simulink model "sm_car"  (R2025a)
settings: Solver=ode23t  StartTime=0.0  StopTime=400  MaxStep=0.4  RelTol=1e-3  AbsTol=1e-3  EnableMultiTasking=on
PreLoadFcn:
  | % Due to usability issue in Repeating Sequence block
  | warning('off','Simulink:Masking:Invalid');
  | 
  | % Eliminate unnecessary warnings in inactive variants
  | % Warnings generated only if you click through inactive variant
  | warning('off','MATLAB:nonExistentField');
  | warning('off','Simulink:Parameters:BlkParamUndefined');
PostLoadFcn:
  | set_param([bdroot '/Vehicle'],'popup_trailer','Off')
  | warning('off','sm:sli:setup:compile:LocalSolverNotSupported')
  | %sm_car_config_maneuver(bdroot,'WOT Braking');
  | sm_car_config_vehicle(bdroot,'false');
  | sm_car_config_logging(bdroot);
InitFcn:
  | sm_car_config_camera;
  | Vehicle = sm_car_vehcfg_checkConfig(Vehicle);
  | sm_car_check_tire_model(bdroot);
StartFcn:
  | tic;
StopFcn:
  | Elapsed_Sim_Time = toc;
  | % disp(['Elapsed Sim Time = ' num2str(Elapsed_Sim_Time)]);
undefined symbols (not defined in the file): Axle1D, AxleIn, Camera, Control, Driver, Free, Init, Maneuver, Pedal, RaceFix, RaceSpin, Scene, ShaftL1, ShaftL2, ShaftR1, ShaftR2, Soft, Stiff, Visual, X, xy_data_car_side, Y, Z
libraries: sm_lib x1546, nesl_utility x528, fl_lib x480, SimscapeFluids_lib x61, sdl_lib x49, simulink x29, ee_lib x7, simulink_extras x6, Linkage_Systems x4, Tire_1x2x x4, AntiRollBar_Systems x2, Linkage_Decoupled x2
(part 19 of 79)

== system sm_car/Vehicle/Vehicle/Chassis/SuspA1/Linkage/Steer ==
  DrvBus : Inport
  CtrlBus : Inport  Port=2
  Wheel Driven Rack 1UJoint : Subsystem  Tag=PublishSubsystem  VariantControl=WheelDrivenRack1UJoint  mask(Steering System with Wheel Actuation){hp_wheel=Steer.Wheel.sMount.Value, wheel_axis_incl=Steer.Wheel.aAxis.Value, hp_mt_rack=Steer.Rack.sMount.Value, hp_out_rack=Steer.Rack.sOutboard.Value, hp_pinion=Steer.Pinion.sMount.Value, Wheel=Steer.Wheel, len_sha_u=Steer.Shaft_Upper.xLength.Value, sha_u_mass=Steer.Shaft_Upper.m.Value, sha_l_mass=Steer.Shaft_Lower.m.Value, rad_pinion=Steer.Pinion.xRad.Value, pinion_mass=Steer.Pinion.m.Value, rack_mass=Steer.Rack.m.Value, whl2steer_filter=1/Steer.Rack.fActuatorCutoff.Value, clr_rack=Visual.SteeringRack.clr, opc_rack=Visual.part.opc, radius_rack=Visual.SteeringRack.rad, clr_shaft=Visual.SteeringShafts.clr, opc_shaft=Visual.part.opc, size_shaft=Visual.SteeringShafts.rad, clr_pinion=Visual.SteeringPinion.clr, opc_pinion=Visual.part.opc, len_pinion=Visual.SteeringPinion.len, clr_connhp=Visual.hp.clr, opc_connhp=Visual.hp.opc, size_connhp=Visual.hp.rad, clr_wheel=Visual.SteeringWheel.clr, opc_wheel=Visual.part.opc, DriverHuman=Steer.DriverHuman}
      mask prompts: hp_wheel "HP Wheel [xyz] (m)"; wheel_axis_incl "Wheel Axis Angle (rad)"; hp_mt_rack "HP Rack Mount [xyz] (m)"; hp_out_rack "HP Track Rod Inboard [xyz] (m)"; hp_pinion "HP Pinion [xyz] (m)"; whl2steer_filter "Steer Motion Filter (sec)"; DriverHuman "Driver Human (structure)"
      mask help: Actuation is applied to steering wheel and transmitted to rack via shafts in steering column. Assumes constant gear ratio between pinion and rack.
      mask init:
      | % Calculate inclination of pinion gear about rack travel axis
      | pinion_incl = atan2(hp_mt_rack(1)-hp_pinion(1),hp_mt_rack(3)-hp_pinion(3));
      | 
      | % Calculate location of universal joint
      | hp_col_upper = hp_wheel  + [+len_sha_u*cos(wheel_axis_incl)  0 -len_sha_u*sin(wheel_axis_incl)];
      mask TypeOptions hp_wheel:
      | Ref to Wheel/Transform
      | HP Wheel/TranslationCartesianOffset
      mask TypeOptions hp_mt_rack:
      | Ref to Rack/Transform
      | HP Rack/TranslationCartesianOffset
      mask TypeOptions hp_out_rack: Rack/hp_out
      mask TypeOptions rack_mass: Rack/rack_mass
      mask TypeOptions whl2steer_filter: Physical Signal/InputFilterTimeConstant
      mask TypeOptions clr_rack: Rack/clr_rack
      mask TypeOptions opc_rack: Rack/opc_rack
      mask TypeOptions radius_rack: Rack/radius_rack
      mask TypeOptions clr_shaft:
      | Shaft
      | Steering/Shaft/GraphicDiffuseColor | Shaft
      | Lower/Shaft/GraphicDiffuseColor | Shaft
      | Intermediate/Shaft/GraphicDiffuseColor
      mask TypeOptions opc_shaft:
      | Shaft
      | Steering/Shaft/GraphicOpacity | Shaft
      | Lower/Shaft/GraphicOpacity | Shaft
      | Intermediate/Shaft/GraphicOpacity
      mask TypeOptions size_shaft:
      | Shaft
      | Steering/Shaft/CylinderRadius | Shaft
      | Lower/Shaft/CylinderRadius | Shaft
      | Intermediate/Shaft/CylinderRadius
      mask TypeOptions clr_pinion: Pinion/Pinion/GraphicDiffuseColor
      mask TypeOptions opc_pinion: Pinion/Pinion/GraphicOpacity
      mask TypeOptions len_pinion: Pinion/Pinion/CylinderLength
      mask TypeOptions clr_connhp:
      | Ref to Rack/Vis
      | Rack
      | Housing/GraphicDiffuseColor | HPs/HP Lower Col/GraphicDiffuseColor | HPs/HP Pinion/GraphicDiffuseColor | HPs/HP Upper Col/GraphicDiffuseColor
      mask TypeOptions opc_connhp:
      | Ref to Rack/Vis
      | Rack
      | Housing/GraphicOpacity | HPs/HP Lower Col/GraphicOpacity | HPs/HP Pinion/GraphicOpacity | HPs/HP Upper Col/GraphicOpacity
      mask TypeOptions size_connhp:
      | Ref to Rack/Vis
      | Rack
      | Housing/SphereRadius | HPs/HP Lower Col/SphereRadius | HPs/HP Pinion/SphereRadius | HPs/HP Upper Col/SphereRadius
      mask TypeOptions clr_wheel: Wheel/clr_wheel
      mask TypeOptions opc_wheel: Wheel/opc_wheel
      mask DialogControl cont_steer Prompt: Steer
      mask DialogControl grp_strparts Prompt: Parts
      mask DialogControl text_strparts_len Prompt: Length/Radius (m)
      mask DialogControl text_strparts_mass Prompt: Mass (kg)
      mask DialogControl text_strparts_wheel Prompt: Wheel
      mask DialogControl text_strparts_wheel_m Prompt: <CAD file>
      mask DialogControl text_strparts_sha_u Prompt: Upper Shaft
      mask DialogControl text_strparts_sha_i Prompt: Lower Shaft
      mask DialogControl text_strparts_sha_i_len Prompt: <length upper, lower>
      mask DialogControl text_strparts_pinion Prompt: Pinion
      mask DialogControl text_strparts_rack Prompt: Rack
      mask DialogControl text_strparts_rack_len Prompt: <HP Rod Inboard>
      mask DialogControl grp_steering Prompt: Steering Input
      mask DialogControl cont_vis_steer Prompt: Visualization
      mask DialogControl text_steer_vis_clr Prompt: Color [RGB]
      mask DialogControl text_steer_vis_opc Prompt: Opac. (0-1)
      mask DialogControl text_steer_vis_size Prompt: Size (m)
      mask DialogControl text_steer_vis_rack Prompt: Rack
      mask DialogControl text_steer_vis_shafts Prompt: Shafts
      mask DialogControl text_steer_vis_pinion Prompt: Pinion
      mask DialogControl text_steer_vis_connhp Prompt: Connections, HP
      mask DialogControl text_steer_vis_wheel Prompt: Wheel
      mask DialogControl text_steer_size_wheel Prompt: <CAD File>
      mask DialogControl cont_driver_human Prompt: Driver Human
  " rodL" : PMIOPort  Side=Right
  " ref" : PMIOPort  Port=2  Side=Right
  " rodR" : PMIOPort  Port=3  Side=Right
  " meas" : Outport  VectorParamsAs1DForOutWhenUnconnected=off

== system sm_car/Vehicle/Vehicle/Chassis/SuspA1/Linkage/Wheel Meas Left ==
  note: For Steering Axis Inclination Estimation
  Bus Creator : BusCreator  Inputs=4
  Calculate Camber : Subsystem
  Calculate Camber Z Axis : Subsystem
  Calculate Toe : Subsystem
  Calculate Toe X Axis : Subsystem
  PS-Simulink Converter1 : nesl_utility/PS-Simulink Converter  PhysicalDomain=network_engine_domain  SubClassName=ps_output  LeftPortType=input  RightPortType=output  PseudoPeriodic=off  Frequencies=[]  VectorFormat=1-D array  Unit=1  AffineConversion=off
  Select x axis : Selector  NumberOfDimensions=2  InputPortWidth=2  IndexOptions=Index vector (dialog),Index vector (dialog)  Indices=[1 2 3],1  OutputSizes=1,1
  Select z axis : Selector  NumberOfDimensions=2  InputPortWidth=2  IndexOptions=Index vector (dialog),Index vector (dialog)  Indices=[1 2 3],3  OutputSizes=1,1
  Sign LR aCamber : Gain  Gain=180/pi*rhs_tc
  Sign LR aCamberX : Gain  Gain=180/pi*rhs_tc
  Sign LR aToe : Gain  Gain=180/pi*rhs_tc
  Sign LR aToeX : Gain  Gain=180/pi*rhs_tc
  Transform Sensor : sm_lib/Frames and Transforms/Transform Sensor  MeasurementFrame=Base  RotationSequence=XYX  SenseAngle=off  SenseAxis=off  SenseQ=off  SenseR=on  SenseRotationSequence=off  SenseOmegaX=off  SenseOmegaY=off  SenseOmegaZ=off  SenseOmega=off  SenseQDot=off  SenseRDot=off  SenseRotationSequenceDot=off  SenseAlphaX=off  SenseAlphaY=off  SenseAlphaZ=off  SenseAlpha=off  SenseQDDot=off  SenseRDDot=off  SenseX=off  SenseY=off  SenseZ=off  SenseXYZ=off  SenseRad=off  SenseAzim=off  SenseDist=off  SenseInc=off  SenseXDot=off  SenseYDot=off  SenseZDot=off  SenseXYZDot=off  SenseRadDot=off  SenseAzimDot=off  SenseDistDot=off  SenseIncDot=off  SenseXDDot=off  SenseYDDot=off  SenseZDDot=off  SenseXYZDDot=off  SenseRadDDot=off  SenseAzimDDot=off  SenseDistDDot=off  SenseIncDDot=off
  Ref : PMIOPort  Side=Left
  Whl Ctr : PMIOPort  Port=2  Side=Left
  meas : Outport  VectorParamsAs1DForOutWhenUnconnected=off
  wires:
  Calculate Toe X Axis/1(Toe) -> Sign LR aToeX/1
  Calculate Camber Z Axis/1(Camber) -> Sign LR aCamberX/1
  Sign LR aCamberX/1 -> Bus Creator/4  "aCamberX"
  Select x axis/1 -> Calculate Toe X Axis/1(uvec spin axis), Calculate Camber Z Axis/1(uvec spin axis)
  Sign LR aToeX/1 -> Bus Creator/3  "aToeX"
  Bus Creator/1 -> meas/1  "Whl"
  Sign LR aToe/1 -> Bus Creator/1  "aToe"
  Sign LR aCamber/1 -> Bus Creator/2  "aCamber"
  PS-Simulink Converter1/1 -> Select x axis/1, Select z axis/1
  Select z axis/1 -> Calculate Camber/1(uvec spin axis), Calculate Toe/1(uvec spin axis)  "uvec spin axis"
  Calculate Camber/1(Camber) -> Sign LR aCamber/1
  Calculate Toe/1(Toe) -> Sign LR aToe/1
  connections:
  Transform Sensor/LConn1 -- Ref/RConn1
  Transform Sensor/RConn1 -- Whl Ctr/RConn1
  PS-Simulink Converter1/LConn1 -- Transform Sensor/RConn2

== system sm_car/Vehicle/Vehicle/Chassis/SuspA1/Linkage/Wheel Meas Right ==
  note: For Steering Axis Inclination Estimation
  Bus Creator : BusCreator  Inputs=4
  Calculate Camber : Subsystem
  Calculate Camber Z Axis : Subsystem
  Calculate Toe : Subsystem
  Calculate Toe X Axis : Subsystem
  PS-Simulink Converter1 : nesl_utility/PS-Simulink Converter  PhysicalDomain=network_engine_domain  SubClassName=ps_output  LeftPortType=input  RightPortType=output  PseudoPeriodic=off  Frequencies=[]  VectorFormat=1-D array  Unit=1  AffineConversion=off
  Select x axis : Selector  NumberOfDimensions=2  InputPortWidth=2  IndexOptions=Index vector (dialog),Index vector (dialog)  Indices=[1 2 3],1  OutputSizes=1,1
  Select z axis : Selector  NumberOfDimensions=2  InputPortWidth=2  IndexOptions=Index vector (dialog),Index vector (dialog)  Indices=[1 2 3],3  OutputSizes=1,1
  Sign LR aCamber : Gain  Gain=180/pi*rhs_tc
  Sign LR aCamberX : Gain  Gain=180/pi*rhs_tc
  Sign LR aToe : Gain  Gain=180/pi*rhs_tc
  Sign LR aToeX : Gain  Gain=180/pi*rhs_tc
  Transform Sensor : sm_lib/Frames and Transforms/Transform Sensor  MeasurementFrame=Base  RotationSequence=XYX  SenseAngle=off  SenseAxis=off  SenseQ=off  SenseR=on  SenseRotationSequence=off  SenseOmegaX=off  SenseOmegaY=off  SenseOmegaZ=off  SenseOmega=off  SenseQDot=off  SenseRDot=off  SenseRotationSequenceDot=off  SenseAlphaX=off  SenseAlphaY=off  SenseAlphaZ=off  SenseAlpha=off  SenseQDDot=off  SenseRDDot=off  SenseX=off  SenseY=off  SenseZ=off  SenseXYZ=off  SenseRad=off  SenseAzim=off  SenseDist=off  SenseInc=off  SenseXDot=off  SenseYDot=off  SenseZDot=off  SenseXYZDot=off  SenseRadDot=off  SenseAzimDot=off  SenseDistDot=off  SenseIncDot=off  SenseXDDot=off  SenseYDDot=off  SenseZDDot=off  SenseXYZDDot=off  SenseRadDDot=off  SenseAzimDDot=off  SenseDistDDot=off  SenseIncDDot=off
  Ref : PMIOPort  Side=Left
  Whl Ctr : PMIOPort  Port=2  Side=Left
  meas : Outport  VectorParamsAs1DForOutWhenUnconnected=off
  wires:
  Calculate Toe X Axis/1(Toe) -> Sign LR aToeX/1
  Calculate Camber Z Axis/1(Camber) -> Sign LR aCamberX/1
  Sign LR aCamberX/1 -> Bus Creator/4  "aCamberX"
  Select x axis/1 -> Calculate Toe X Axis/1(uvec spin axis), Calculate Camber Z Axis/1(uvec spin axis)
  Sign LR aToeX/1 -> Bus Creator/3  "aToeX"
  Bus Creator/1 -> meas/1  "Whl"
  Sign LR aToe/1 -> Bus Creator/1  "aToe"
  Sign LR aCamber/1 -> Bus Creator/2  "aCamber"
  PS-Simulink Converter1/1 -> Select x axis/1, Select z axis/1
  Select z axis/1 -> Calculate Camber/1(uvec spin axis), Calculate Toe/1(uvec spin axis)  "uvec spin axis"
  Calculate Camber/1(Camber) -> Sign LR aCamber/1
  Calculate Toe/1(Toe) -> Sign LR aToe/1
  connections:
  Transform Sensor/LConn1 -- Ref/RConn1
  Transform Sensor/RConn1 -- Whl Ctr/RConn1
  PS-Simulink Converter1/LConn1 -- Transform Sensor/RConn2

== system sm_car/Vehicle/Vehicle/Chassis/SuspA1/Linkage Decoupled/RollHeave Decouple ==
  HP Heave L : Subsystem  mask(Revolute Joint 3 Points){popup_leftRight=Left, hp_bcr_pivot=hp_bcr_pivot, hp_pushrod_in=hp_pushrod, hp_bcr_shock=hp_bcr_shock_heaveL}
      mask prompts: popup_leftRight "Left/Right"; hp_bcr_pivot "HP Bellcrank Pivot [xyz] (m)"; hp_pushrod_in "HP Pushrod Inner [xyz] (m)"; hp_bcr_shock "HP Bellcrank Shock Heave [xyz] (m)"
      mask help: Revolute Joint with degree of freedom normal to 3 hardpoints.
      mask init:
      | % Set parameter for mirroring (+y or -y)
      | if(popup_leftRight == 1)
      |     rhs_susp = 1;    
      | elseif(popup_leftRight == 2)
      |     rhs_susp = -1;
      | end
      | 
      | rhs_hp = [1 rhs_susp 1];
      mask TypeOptions popup_leftRight: Left | Right
      mask Display: image('sm_car_variant_revolute.png')
  HP HeaveR : Subsystem  mask(Revolute Joint 3 Points){popup_leftRight=Right, hp_bcr_pivot=hp_bcr_pivot, hp_pushrod_in=hp_pushrod, hp_bcr_shock=hp_bcr_shock_heaveR}
      mask prompts: popup_leftRight "Left/Right"; hp_bcr_pivot "HP Bellcrank Pivot [xyz] (m)"; hp_pushrod_in "HP Pushrod Inner [xyz] (m)"; hp_bcr_shock "HP Bellcrank Shock Heave [xyz] (m)"
      mask help: Revolute Joint with degree of freedom normal to 3 hardpoints.
      mask init:
      | % Set parameter for mirroring (+y or -y)
      | if(popup_leftRight == 1)
      |     rhs_susp = 1;    
      | elseif(popup_leftRight == 2)
      |     rhs_susp = -1;
      | end
      | 
      | rhs_hp = [1 rhs_susp 1];
      mask TypeOptions popup_leftRight: Left | Right
      mask Display: image('sm_car_variant_revolute.png')
  HP Roll L : Subsystem  mask(Revolute Joint 3 Points){popup_leftRight=Left, hp_bcr_pivot=hp_bcr_pivot, hp_pushrod_in=hp_pushrod, hp_bcr_shock=hp_bcr_shock_heaveL}
      mask prompts: popup_leftRight "Left/Right"; hp_bcr_pivot "HP Bellcrank Pivot [xyz] (m)"; hp_pushrod_in "HP Pushrod Inner [xyz] (m)"; hp_bcr_shock "HP Bellcrank Shock Heave [xyz] (m)"
      mask help: Revolute Joint with degree of freedom normal to 3 hardpoints.
      mask init:
      | % Set parameter for mirroring (+y or -y)
      | if(popup_leftRight == 1)
      |     rhs_susp = 1;    
      | elseif(popup_leftRight == 2)
      |     rhs_susp = -1;
      | end
      | 
      | rhs_hp = [1 rhs_susp 1];
      mask TypeOptions popup_leftRight: Left | Right
      mask Display: image('sm_car_variant_revolute.png')
  HP Roll R : Subsystem  mask(Revolute Joint 3 Points){popup_leftRight=Right, hp_bcr_pivot=hp_bcr_pivot, hp_pushrod_in=hp_pushrod, hp_bcr_shock=hp_bcr_shock_heaveR}
      mask prompts: popup_leftRight "Left/Right"; hp_bcr_pivot "HP Bellcrank Pivot [xyz] (m)"; hp_pushrod_in "HP Pushrod Inner [xyz] (m)"; hp_bcr_shock "HP Bellcrank Shock Heave [xyz] (m)"
      mask help: Revolute Joint with degree of freedom normal to 3 hardpoints.
      mask init:
      | % Set parameter for mirroring (+y or -y)
      | if(popup_leftRight == 1)
      |     rhs_susp = 1;    
      | elseif(popup_leftRight == 2)
      |     rhs_susp = -1;
      | end
      | 
      | rhs_hp = [1 rhs_susp 1];
      mask TypeOptions popup_leftRight: Left | Right
      mask Display: image('sm_car_variant_revolute.png')
  PS-Simulink Converter{,1..3} (4 alike) : nesl_utility/PS-Simulink Converter  PhysicalDomain=network_engine_domain  SubClassName=ps_output  LeftPortType=input  RightPortType=output  PseudoPeriodic=off  Frequencies=[]  VectorFormat=1-D array  Unit=1  AffineConversion=off
  Shock Heave : Subsystem  mask{shock_pist_mass=shock_pist_mass_heave, shock_cyl_mass=shock_cyl_mass_heave, hp_spr_top=hp_bcr_shock_heaveR, hp_spr_bot=hp_bcr_shock_heaveL, up_lim_bumpstop=up_lim_bumpstop_heave, low_lim_bumpstop=low_lim_bumpstop_heave, clr_conn_shock=clr_conn_shock, opc_conn_shock=opc_conn_shock, size_conn_shock=size_conn_shock, clr_shock_cyl=clr_shock_cyl, opc_shock_cyl=opc_shock_cyl, radius_shock_cyl=radius_shock_cyl, clr_shock_piston=clr_shock_piston, opc_shock_piston=opc_shock_piston, clr_shock_bumpstop=clr_shock_bumpstop, opc_shock_bumpstop=opc_shock_bumpstop, deadvol_len_shock_cyl=deadvol_len_shock_cyl, piston_len_shock=piston_len_shock, cyl_cap_len_shock=cyl_cap_len_shock, bumpstop_len_shock=bumpstop_len_shock}
      mask prompts: shock_pist_mass "Piston Mass (kg)"; shock_cyl_mass "Cylinder Mass (kg)"; hp_spr_top "Shock Top [xyz] (m)"; hp_spr_bot "Shock Bottom [xyz] (m)"; up_lim_bumpstop "Upper Limit Bumpstop (m)"; low_lim_bumpstop "Lower Limit Bumpstop (m)"; deadvol_len_shock_cyl "Dead Volume Height (m)"; piston_len_shock "Piston Length (m)"; cyl_cap_len_shock "Cylinder Cap Length (m)"; bumpstop_len_shock "Bumpstop Length (m)"
      mask init:
      | init_spr_len = norm(hp_spr_top-hp_spr_bot);
      | 
      | rod_length_upper = ...
      | cyl_cap_len_shock + bumpstop_len_shock + abs(low_lim_bumpstop) + ...
      | cyl_cap_len_shock + abs(up_lim_bumpstop) + piston_len_shock;
      | 
      | rod_length_lower = init_spr_len - rod_length_upper - deadvol_len_shock_cyl - cyl_cap_len_shock - abs(low_lim_bumpstop);
      | 
      | bumpstop_xc_rev = [0 0; 0.7 0; 0.9 1; 0 1].*[radius_shock_cyl bumpstop_len_shock];
      | 
      | cyl_wall_length = piston_len_shock+abs(low_lim_bumpstop)+abs(up_lim_bumpstop)+deadvol_len_shock_cyl;
      mask Help: web('sm_car_doc_susp_shock.html')
      mask TypeOptions shock_pist_mass: Piston/Rod/Mass
      mask TypeOptions shock_cyl_mass: Cylinder/Wall/Mass
      mask TypeOptions clr_conn_shock:
      | Vis
      | HP L/GraphicDiffuseColor | Vis
      | HP U/GraphicDiffuseColor
      mask TypeOptions opc_conn_shock:
      | Vis
      | HP L/GraphicOpacity | Vis
      | HP U/GraphicOpacity
      mask TypeOptions clr_shock_cyl: Cylinder/Cap Bottom/GraphicDiffuseColor | Cylinder/Cap Top/GraphicDiffuseColor | Cylinder/Wall/GraphicDiffuseColor
      mask TypeOptions clr_shock_piston: Piston/Cap/GraphicDiffuseColor | Piston/Piston/GraphicDiffuseColor | Piston/Rod/GraphicDiffuseColor
      mask TypeOptions opc_shock_piston: Piston/Cap/GraphicOpacity | Piston/Piston/GraphicOpacity | Piston/Rod/GraphicOpacity
      mask TypeOptions clr_shock_bumpstop: Piston/Bumpstop/GraphicDiffuseColor
      mask TypeOptions opc_shock_bumpstop: Piston/Bumpstop/GraphicOpacity
      mask DialogControl cont_shock Prompt: Shock
      mask DialogControl cont_vis_shock Prompt: Visualization
      mask DialogControl text_blank_shock Prompt: (Add text here)
      mask DialogControl text_clr_shock Prompt: Color  [RGB]
      mask DialogControl text_opc_shock Prompt: Opac. (0-1)
      mask DialogControl text_size_shock Prompt: Size (m)
      mask DialogControl text_conn_shock Prompt: Connections
      mask DialogControl text_shock_cyl Prompt: Cylinder
      mask DialogControl text_shock_piston Prompt: Piston
      mask DialogControl text_piston_radius Prompt: <cylinder radius>
      mask DialogControl text_shock_bumpstop Prompt: Bumpstop
      mask DialogControl text_bumpstop_radius Prompt: <cylinder radius>
      mask Display: image('sm_car_vehicle_linkage_shock_hpu_IMAGE.png');
  Shock Roll : Subsystem  mask{shock_pist_mass=shock_pist_mass_roll, shock_cyl_mass=shock_cyl_mass_roll, hp_spr_top=hp_bcr_shock_rollR, hp_spr_bot=hp_bcr_shock_rollL, up_lim_bumpstop=up_lim_bumpstop_roll, low_lim_bumpstop=low_lim_bumpstop_roll, clr_conn_shock=clr_conn_shock, opc_conn_shock=opc_conn_shock, size_conn_shock=size_conn_shock, clr_shock_cyl=clr_shock_cyl, opc_shock_cyl=opc_shock_cyl, radius_shock_cyl=radius_shock_cyl, clr_shock_piston=clr_shock_piston, opc_shock_piston=opc_shock_piston, clr_shock_bumpstop=clr_shock_bumpstop, opc_shock_bumpstop=opc_shock_bumpstop, deadvol_len_shock_cyl=deadvol_len_shock_cyl, piston_len_shock=piston_len_shock, cyl_cap_len_shock=cyl_cap_len_shock, bumpstop_len_shock=bumpstop_len_shock}
      mask prompts: shock_pist_mass "Piston Mass (kg)"; shock_cyl_mass "Cylinder Mass (kg)"; hp_spr_top "Shock Top [xyz] (m)"; hp_spr_bot "Shock Bottom [xyz] (m)"; up_lim_bumpstop "Upper Limit Bumpstop (m)"; low_lim_bumpstop "Lower Limit Bumpstop (m)"; deadvol_len_shock_cyl "Dead Volume Height (m)"; piston_len_shock "Piston Length (m)"; cyl_cap_len_shock "Cylinder Cap Length (m)"; bumpstop_len_shock "Bumpstop Length (m)"
      mask init: same as sm_car/Vehicle/Vehicle/Chassis/SuspA1/Linkage Decoupled/RollHeave Decouple/Shock Heave
      mask Help: web('sm_car_doc_susp_shock.html')
      mask TypeOptions shock_pist_mass: Piston/Rod/Mass
      mask TypeOptions shock_cyl_mass: Cylinder/Wall/Mass
      mask TypeOptions clr_conn_shock:
      | Vis
      | HP L/GraphicDiffuseColor | Vis
      | HP U/GraphicDiffuseColor
      mask TypeOptions opc_conn_shock:
      | Vis
      | HP L/GraphicOpacity | Vis
      | HP U/GraphicOpacity
      mask TypeOptions clr_shock_cyl: Cylinder/Cap Bottom/GraphicDiffuseColor | Cylinder/Cap Top/GraphicDiffuseColor | Cylinder/Wall/GraphicDiffuseColor
      mask TypeOptions clr_shock_piston: Piston/Cap/GraphicDiffuseColor | Piston/Piston/GraphicDiffuseColor | Piston/Rod/GraphicDiffuseColor
      mask TypeOptions opc_shock_piston: Piston/Cap/GraphicOpacity | Piston/Piston/GraphicOpacity | Piston/Rod/GraphicOpacity
      mask TypeOptions clr_shock_bumpstop: Piston/Bumpstop/GraphicDiffuseColor
      mask TypeOptions opc_shock_bumpstop: Piston/Bumpstop/GraphicOpacity
      mask DialogControl cont_shock Prompt: Shock
      mask DialogControl cont_vis_shock Prompt: Visualization
      mask DialogControl text_blank_shock Prompt: (Add text here)
      mask DialogControl text_clr_shock Prompt: Color  [RGB]
      mask DialogControl text_opc_shock Prompt: Opac. (0-1)
      mask DialogControl text_size_shock Prompt: Size (m)
      mask DialogControl text_conn_shock Prompt: Connections
      mask DialogControl text_shock_cyl Prompt: Cylinder
      mask DialogControl text_shock_piston Prompt: Piston
      mask DialogControl text_piston_radius Prompt: <cylinder radius>
      mask DialogControl text_shock_bumpstop Prompt: Bumpstop
      mask DialogControl text_bumpstop_radius Prompt: <cylinder radius>
      mask Display: image('sm_car_vehicle_linkage_shock_hpu_IMAGE.png');
  Transform Align Axis 2P HeaveL : Subsystem  mask(Transform Align Axis Two Points){hp_b=hp_bcr_shock_heaveL, hp_t=hp_bcr_shock_heaveR, popup_f_axis=+Z}
      mask prompts: hp_b "Location of B [xyz] (m)"; hp_t "Target for Frame Axis [xyz] (m)"; popup_f_axis "Axis of F Frame to Aim at Target"
      mask help: Transforms a frame to aim a selected axis at a target point. Both points must be defined relative to the same reference frame.
      mask init:
      | switch popup_f_axis
      |     case 1, vec = [ 1  0  0];
      |     case 2, vec = [ 0  1  0];
      |     case 3, vec = [ 0  0  1];
      |     case 4, vec = [-1  0  0];
      |     case 5, vec = [ 0 -1  0];
      |     case 6, vec = [ 0  0 -1];
      | end
      | 
      | uvec_bt = (hp_t-hp_b)/norm(hp_t-hp_b);
      | rotaxis = cross(vec,uvec_bt);
      | 
      | if (norm(rotaxis)==0)
      |     if (uvec_bt==0)            % hps collocated
      |         rotangle = 0; 
      |     elseif ((uvec_bt+vec)==0)  % vectors antiparallel    
      |         rotangle = pi;
      |         rotaxis = circshift(vec,1);
      |     else                       % vectors parallel
      |         rotangle = 0;          
      |     end
      | else
      |     rotangle = acos(dot(vec,uvec_bt));
      |     %rotangle = acos(dot(vec,(hp_t-hp_b)/norm((hp_t-hp_b))))
      | end
      mask TypeOptions popup_f_axis: +X | +Y | +Z | -X | -Y | -Z
      mask Display: image('sm_car_transform_align_axis_two_points.png')
  Transform Align Axis 2P HeaveR : Subsystem  mask(Transform Align Axis Two Points){hp_b=hp_bcr_shock_heaveR, hp_t=hp_bcr_shock_heaveL, popup_f_axis=-Z}
      mask prompts: hp_b "Location of B [xyz] (m)"; hp_t "Target for Frame Axis [xyz] (m)"; popup_f_axis "Axis of F Frame to Aim at Target"
      mask help: Transforms a frame to aim a selected axis at a target point. Both points must be defined relative to the same reference frame.
      mask init: same as sm_car/Vehicle/Vehicle/Chassis/SuspA1/Linkage Decoupled/RollHeave Decouple/Transform Align Axis 2P HeaveL
      mask TypeOptions popup_f_axis: +X | +Y | +Z | -X | -Y | -Z
      mask Display: image('sm_car_transform_align_axis_two_points.png')
  Transform Align Axis 2P RollL : Subsystem  mask(Transform Align Axis Two Points){hp_b=hp_bcr_shock_rollL, hp_t=hp_bcr_shock_rollR, popup_f_axis=+Z}
      mask prompts: hp_b "Location of B [xyz] (m)"; hp_t "Target for Frame Axis [xyz] (m)"; popup_f_axis "Axis of F Frame to Aim at Target"
      mask help: Transforms a frame to aim a selected axis at a target point. Both points must be defined relative to the same reference frame.
      mask init: same as sm_car/Vehicle/Vehicle/Chassis/SuspA1/Linkage Decoupled/RollHeave Decouple/Transform Align Axis 2P HeaveL
      mask TypeOptions popup_f_axis: +X | +Y | +Z | -X | -Y | -Z
      mask Display: image('sm_car_transform_align_axis_two_points.png')
  Transform Align Axis 2P RollR : Subsystem  mask(Transform Align Axis Two Points){hp_b=hp_bcr_shock_rollR, hp_t=hp_bcr_shock_rollL, popup_f_axis=-Z}
      mask prompts: hp_b "Location of B [xyz] (m)"; hp_t "Target for Frame Axis [xyz] (m)"; popup_f_axis "Axis of F Frame to Aim at Target"
      mask help: Transforms a frame to aim a selected axis at a target point. Both points must be defined relative to the same reference frame.
      mask init: same as sm_car/Vehicle/Vehicle/Chassis/SuspA1/Linkage Decoupled/RollHeave Decouple/Transform Align Axis 2P HeaveL
      mask TypeOptions popup_f_axis: +X | +Y | +Z | -X | -Y | -Z
      mask Display: image('sm_car_transform_align_axis_two_points.png')
  "Transform HP Heave L " : sm_lib/Frames and Transforms/Rigid Transform  RotationMethod=None  FollAlignAxisA=+X  BaseAlignAxisA=+Y  FollAlignAxisB=+Y  BaseAlignAxisB=+Z  RotationStandardAxis=+Z  RotationAngle=0.0  RotationAngleUnits=deg  RotationArbitraryAxis=[0 0 1]  RotationSequenceAxes=FollowerAxes  RotationSequence=XYX  RotationSequenceAngles=[0 0 0]  RotationSequenceAnglesUnits=deg  RotationMatrix=[1 0 0; 0 1 0; 0 0 1]  Quaternion=[1 0 0 0]  TranslationMethod=Cartesian  TranslationCartesianOffset=hp_bcr_shock_heaveL  TranslationCartesianOffsetUnits=m  TranslationStandardAxis=+Z  TranslationStandardOffset=0  TranslationStandardOffsetUnits=m  TranslationROffset=0  TranslationROffsetUnits=m  TranslationThetaOffset=0  TranslationThetaOffsetUnits=deg  TranslationZOffset=0  TranslationZOffsetUnits=m
  Transform HP Heave R : sm_lib/Frames and Transforms/Rigid Transform  RotationMethod=None  FollAlignAxisA=+X  BaseAlignAxisA=+Y  FollAlignAxisB=+Y  BaseAlignAxisB=+Z  RotationStandardAxis=+Z  RotationAngle=0.0  RotationAngleUnits=deg  RotationArbitraryAxis=[0 0 1]  RotationSequenceAxes=FollowerAxes  RotationSequence=XYX  RotationSequenceAngles=[0 0 0]  RotationSequenceAnglesUnits=deg  RotationMatrix=[1 0 0; 0 1 0; 0 0 1]  Quaternion=[1 0 0 0]  TranslationMethod=Cartesian  TranslationCartesianOffset=hp_bcr_shock_heaveR  TranslationCartesianOffsetUnits=m  TranslationStandardAxis=+Z  TranslationStandardOffset=0  TranslationStandardOffsetUnits=m  TranslationROffset=0  TranslationROffsetUnits=m  TranslationThetaOffset=0  TranslationThetaOffsetUnits=deg  TranslationZOffset=0  TranslationZOffsetUnits=m
  Transform HP Roll L : sm_lib/Frames and Transforms/Rigid Transform  RotationMethod=None  FollAlignAxisA=+X  BaseAlignAxisA=+Y  FollAlignAxisB=+Y  BaseAlignAxisB=+Z  RotationStandardAxis=+Z  RotationAngle=0.0  RotationAngleUnits=deg  RotationArbitraryAxis=[0 0 1]  RotationSequenceAxes=FollowerAxes  RotationSequence=XYX  RotationSequenceAngles=[0 0 0]  RotationSequenceAnglesUnits=deg  RotationMatrix=[1 0 0; 0 1 0; 0 0 1]  Quaternion=[1 0 0 0]  TranslationMethod=Cartesian  TranslationCartesianOffset=hp_bcr_shock_rollL  TranslationCartesianOffsetUnits=m  TranslationStandardAxis=+Z  TranslationStandardOffset=0  TranslationStandardOffsetUnits=m  TranslationROffset=0  TranslationROffsetUnits=m  TranslationThetaOffset=0  TranslationThetaOffsetUnits=deg  TranslationZOffset=0  TranslationZOffsetUnits=m
  Transform HP Roll R : sm_lib/Frames and Transforms/Rigid Transform  RotationMethod=None  FollAlignAxisA=+X  BaseAlignAxisA=+Y  FollAlignAxisB=+Y  BaseAlignAxisB=+Z  RotationStandardAxis=+Z  RotationAngle=0.0  RotationAngleUnits=deg  RotationArbitraryAxis=[0 0 1]  RotationSequenceAxes=FollowerAxes  RotationSequence=XYX  RotationSequenceAngles=[0 0 0]  RotationSequenceAnglesUnits=deg  RotationMatrix=[1 0 0; 0 1 0; 0 0 1]  Quaternion=[1 0 0 0]  TranslationMethod=Cartesian  TranslationCartesianOffset=hp_bcr_shock_rollR  TranslationCartesianOffsetUnits=m  TranslationStandardAxis=+Z  TranslationStandardOffset=0  TranslationStandardOffsetUnits=m  TranslationROffset=0  TranslationROffsetUnits=m  TranslationThetaOffset=0  TranslationThetaOffsetUnits=deg  TranslationZOffset=0  TranslationZOffsetUnits=m
  SHL : PMIOPort  Side=Left
  SRL : PMIOPort  Port=2  Side=Left
  SH : PMIOPort  Port=3  Side=Left
  DH : PMIOPort  Port=4  Side=Left
  DR : PMIOPort  Port=5  Side=Left
  SR : PMIOPort  Port=6  Side=Left
  SRR : PMIOPort  Port=7  Side=Left
  SHR : PMIOPort  Port=8  Side=Left
  Out Bus Element : Outport  VectorParamsAs1DForOutWhenUnconnected=off  PortName=meas  Element=qHL
  Out Bus Element3 : Outport  VectorParamsAs1DForOutWhenUnconnected=off  PortName=meas  Element=qHR
  Out Bus Element1 : Outport  VectorParamsAs1DForOutWhenUnconnected=off  PortName=meas  Element=qRL
  Out Bus Element2 : Outport  VectorParamsAs1DForOutWhenUnconnected=off  PortName=meas  Element=qRR
  Out Bus Element4 : Outport  VectorParamsAs1DForOutWhenUnconnected=off  PortName=meas  Element=xHeave
  Out Bus Element5 : Outport  VectorParamsAs1DForOutWhenUnconnected=off  PortName=meas  Element=xRoll
  wires:
  Shock Roll/1(m) -> Out Bus Element5/1
  Shock Heave/1(m) -> Out Bus Element4/1
  PS-Simulink Converter3/1 -> Out Bus Element2/1
  PS-Simulink Converter2/1 -> Out Bus Element3/1
  PS-Simulink Converter1/1 -> Out Bus Element/1
  PS-Simulink Converter/1 -> Out Bus Element1/1
  connections:
  PS-Simulink Converter3/LConn1 -- HP Roll R/RConn2
  PS-Simulink Converter2/LConn1 -- HP HeaveR/RConn2
  PS-Simulink Converter1/LConn1 -- HP Heave L/RConn2
  PS-Simulink Converter/LConn1 -- HP Roll L/RConn2
  HP Heave L/RConn1 -- Transform Align Axis 2P HeaveL/LConn1
  Shock Heave/RConn2 -- Transform Align Axis 2P HeaveR/RConn1
  Shock Roll/LConn1 -- Transform Align Axis 2P RollL/RConn1
  Shock Roll/RConn2 -- Transform Align Axis 2P RollR/RConn1
  HP Roll R/LConn1 -- Transform HP Roll R/RConn1
  HP Roll L/LConn1 -- Transform HP Roll L/RConn1
  Transform HP Roll L/LConn1 -- SRL/RConn1
  HP Roll L/RConn1 -- Transform Align Axis 2P RollL/LConn1
  Transform HP Roll R/LConn1 -- SRR/RConn1
  HP Roll R/RConn1 -- Transform Align Axis 2P RollR/LConn1
  Shock Roll/RConn1 -- SR/RConn1 -- DR/RConn1
  DH/RConn1 -- Shock Heave/RConn1 -- SH/RConn1
  HP Heave L/LConn1 -- "Transform HP Heave L "/RConn1
  HP HeaveR/RConn1 -- Transform Align Axis 2P HeaveR/LConn1
  HP HeaveR/LConn1 -- Transform HP Heave R/RConn1
  Transform HP Heave R/LConn1 -- SHR/RConn1
  Transform Align Axis 2P HeaveL/RConn1 -- Shock Heave/LConn1
  "Transform HP Heave L "/LConn1 -- SHL/RConn1
